simulink model "CMSD_Evaluation"  (R2024b)
settings: Solver=ode45  StartTime=0.0  StopTime=60  MaxStep=0.01  MinStep=0.01  RelTol=1e-3
undefined symbols (not defined in the file or in its folder): ref_seed
libraries: simulink x1, rllib x1
settings Model: Creator=minhh  LastModifiedBy=minhh
settings SolverCC: InitialStep=0.01

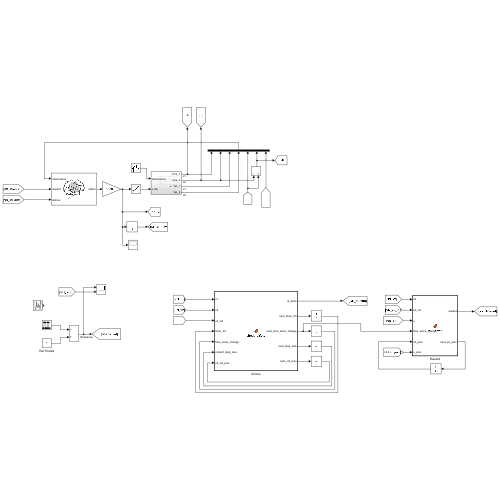
[thumbnail: Simulink's stored preview of the top-level diagram]
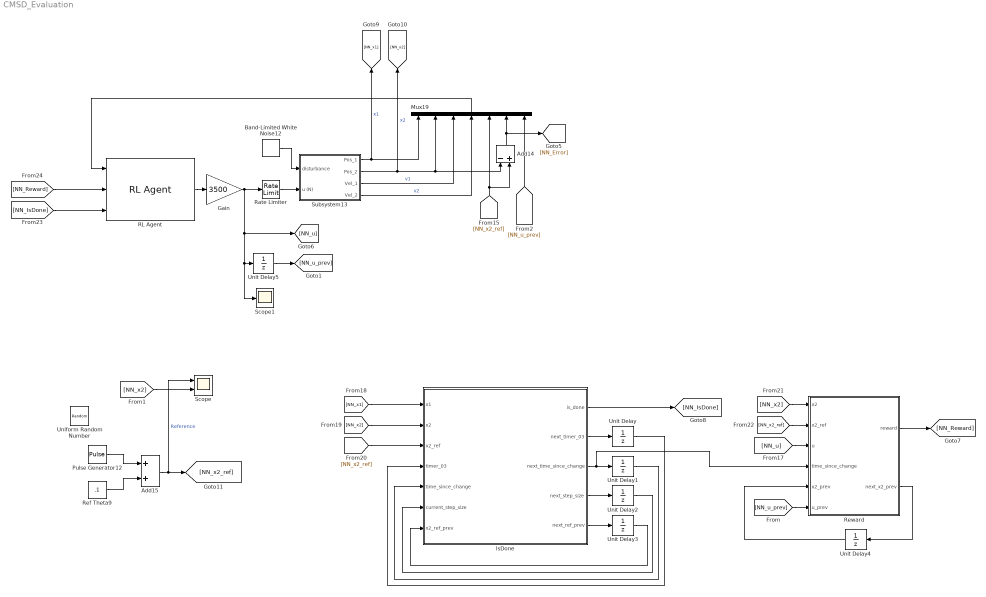
== system CMSD_Evaluation ==
  Add14 : Sum  Inputs=-+
  Add15 : Sum
  Band-Limited White Noise12 : simulink/Sources/Band-Limited White Noise  Cov=[200]  Ts=0.01  seed=[23341]
  Gain : Gain  Gain=3500
  IsDone : MATLAB Function  TreatAsAtomicUnit=on
  Mux19 : Mux  Inputs=7
  Pulse Generator12 : DiscretePulseGenerator  Amplitude=0.3  Period=10000  PulseWidth=2000  PhaseDelay=2000  SampleTime=0.01
  RL Agent : rllib/RL Agent  Agent=agentObj  ExternalActionAsInput=off  ProvideLastAction=off  ProvideCumRwd=off  TreatAsDirectFeedthrough=on  UseStrictObservationDataTypes=off
  Rate Limiter : RateLimiter  RisingSlewLimit=25000  FallingSlewLimit=-25000  SampleTimeMode=inherited
  Ref Theta9 : Constant  Value=.1  SampleTime=0.01
  Reward : MATLAB Function  TreatAsAtomicUnit=on
  Scope : Scope  NumInputPorts=2
  Scope1 : Scope
  Subsystem13 : Subsystem
  Uniform Random Number : UniformRandomNumber  Minimum=-0.2  Maximum=0.5  Seed=ref_seed  SampleTime=8
  Unit Delay{,1..5} (6 alike) : UnitDelay  SampleTime=0.01  HasFrameUpgradeWarning=on
  wires:
  [NN_IsDone] -> RL Agent/3
  [NN_x2] -> Reward/1(x2)
  IsDone/1(is_done) -> [NN_IsDone]
  Unit Delay3/1 -> IsDone/7(x2_ref_prev)
  Rate Limiter/1 -> Subsystem13/2(u (N))
  [NN_x2_ref] -> Mux19/5, Add14/2
  Unit Delay2/1 -> IsDone/6(current_step_size)
  IsDone/5(next_ref_prev) -> Unit Delay3/1
  [NN_x2_ref] -> IsDone/3(x2_ref)
  IsDone/2(next_timer_03) -> Unit Delay/1
  IsDone/3(next_time_since_change) -> Reward/4(time_since_change), Unit Delay1/1
  Unit Delay4/1 -> Reward/5(x2_prev)
  [NN_x2] -> IsDone/2(x2)
  Band-Limited White Noise12/1 -> Subsystem13/1(disturbance)
  Subsystem13/2(Pos_2) -> Add14/1, Mux19/2, [NN_x2]  "x2"
  [NN_u] -> Reward/3(u)
  IsDone/4(next_step_size) -> Unit Delay2/1
  Subsystem13/3(Vel_1) -> Mux19/3  "v1"
  [NN_Reward] -> RL Agent/2
  Reward/1(reward) -> [NN_Reward]
  [NN_x1] -> IsDone/1(x1)
  Unit Delay/1 -> IsDone/4(timer_03)
  Subsystem13/4(Vel_2) -> Mux19/4  "v2"
  [NN_x2_ref] -> Reward/2(x2_ref)
  Unit Delay1/1 -> IsDone/5(time_since_change)
  Gain/1 -> Scope1/1, Unit Delay5/1, [NN_u], Rate Limiter/1
  Reward/2(next_x2_prev) -> Unit Delay4/1
  Mux19/1 -> RL Agent/1
  Add14/1 -> [NN_Error], Mux19/6
  [NN_u_prev] -> Reward/6(u_prev)
  Unit Delay5/1 -> [NN_u_prev]
  Subsystem13/1(Pos_1) -> Mux19/1, [NN_x1]  "x1"
  RL Agent/1 -> Gain/1
  Pulse Generator12/1 -> Add15/1
  Ref Theta9/1 -> Add15/2
  [NN_x2] -> Scope/2
  Add15/1 -> Scope/1, [NN_x2_ref]  "Reference"
  [NN_u_prev] -> Mux19/7

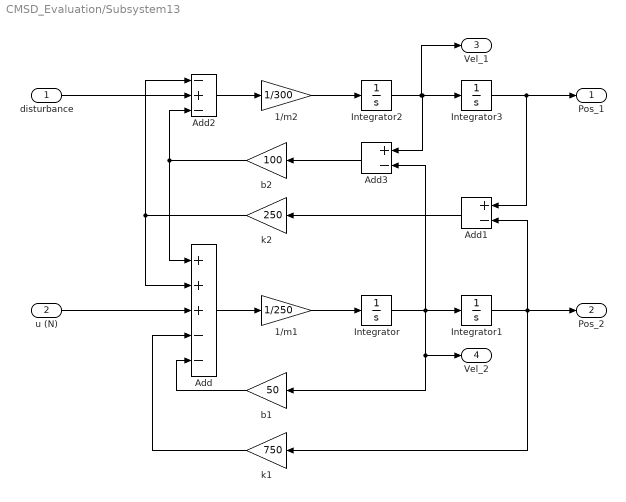
== system CMSD_Evaluation/Subsystem13 ==
  disturbance : Inport
  u (N) : Inport  Port=2
  1/m1 : Gain  Gain=1/250
  1/m2 : Gain  Gain=1/300
  Add : Sum  Inputs=+++--
  Add1 : Sum  Inputs=+-
  Add2 : Sum  Inputs=-+-
  Add3 : Sum  Inputs=+-
  Integrator{,1..3} (4 alike) : Integrator
  b1 : Gain  Gain=50
  b2 : Gain  Gain=100
  k1 : Gain  Gain=750
  k2 : Gain  Gain=250
  Pos_1 : Outport
  Pos_2 : Outport  Port=2
  Vel_1 : Outport  Port=3
  Vel_2 : Outport  Port=4
  wires:
  Add/1 -> 1/m1/1
  1/m1/1 -> Integrator/1
  Integrator/1 -> Add3/2, Integrator1/1, b1/1, Vel_2/1
  Integrator1/1 -> k1/1, Pos_2/1, Add1/2
  Add2/1 -> 1/m2/1
  1/m2/1 -> Integrator2/1
  Integrator2/1 -> Vel_1/1, Add3/1, Integrator3/1
  Add3/1 -> b2/1
  b2/1 -> Add2/3, Add/1
  Add1/1 -> k2/1
  Integrator3/1 -> Pos_1/1, Add1/1
  u (N)/1 -> Add/3
  b1/1 -> Add/5
  k1/1 -> Add/4
  k2/1 -> Add2/1, Add/2
  disturbance/1 -> Add2/2

== matlab function CMSD_Evaluation/Reward ==
  data: x2 input; x2_ref input; u input; reward output; time_since_change input; x2_prev input; next_x2_prev output; u_prev input
function [reward, next_x2_prev] = calc_reward(x2, x2_ref, u, time_since_change, x2_prev, u_prev)
    
    % --- ENFORCE STRICT DATA TYPES FOR COMPILER ---
    reward = double(0.1); 
    next_x2_prev = double(x2); 
    
    x2_error = double(abs(x2_ref - x2));
    delta_x2 = double(abs(x2 - x2_prev));
    delta_u  = double(abs(u - u_prev));
    
    % --- 1. TIGHT BOUNDARY BLEED (0.0050m) ---
    reward = double(reward - (10.0 * x2_error^2)); 
    
    if x2_error > 0.0050
        reward = double(reward - 1.0); 
    else
        reward = double(reward + 2.0); 
    end
    
    % --- 2. SMC ROBUSTNESS (Settle-Time Grace Period) ---
    if time_since_change > 1.0
        if delta_x2 > 0.005
            reward = double(reward - 5.0); 
        end
    end
    
    % --- 3. ENERGY EFFICIENCY ---
    reward = double(reward - 0.5 * ((u / 3500.0)^2));
    
    % --- 4. HARDWARE LIMIT PENALTY (250N/step) ---
    if delta_u > 500.0
        violation = double(delta_u - 500.0);
        reward = double(reward - (violation^2)); 
    end

    % --- THE ANTI-SUICIDE PATCH ---
    % If the AI violently jerks the motor and breaks the x1 limit, 
    % it receives a penalty so massive it will never do it again.
    if abs(x1) > 0.65
        reward = double(reward - 6000.0);
    end
    
end

== matlab function CMSD_Evaluation/IsDone ==
  data: x1 input; is_done output; x2 input; x2_ref input; next_timer_03 output; timer_03 input; time_since_change input; current_step_size input; x2_ref_prev input; next_time_since_change output; next_step_size output; next_ref_prev output
function [is_done, next_timer_03, next_time_since_change, next_step_size, next_ref_prev] = check_safety(x1, x2, x2_ref, timer_03, time_since_change, current_step_size, x2_ref_prev)
    
    % --- ENFORCE STRICT DATA TYPES FOR THE COMPILER ---
    is_done = double(0); % <--- Changed to double(0) instead of false
    next_timer_03 = double(timer_03);
    next_time_since_change = double(time_since_change);
    next_step_size = double(current_step_size);
    next_ref_prev = double(x2_ref_prev);
    
    dt = double(0.01); 
    x2_error = double(x2_ref - x2);
    
    % --- 1. DETECT A REFERENCE CHANGE ---
    if abs(x2_ref - x2_ref_prev) > 0.001
        next_time_since_change = double(0.0);
        next_step_size = double(abs(x2_ref - x2_ref_prev));
    else
        next_time_since_change = double(time_since_change + dt);
    end
    next_ref_prev = double(x2_ref);
    
    % --- 2. DEATH CONDITIONS ---
    if abs(x1) > 0.65
        is_done = double(1); % <--- Changed to double(1) instead of true
    end
    
% --- RELAXED DEATH CONDITIONS FOR CURRICULUM LEARNING ---
    
    % Give it 3.0 seconds to fix a massive error instead of 0.75s
    if abs(x2_error) > 0.3
        next_timer_03 = double(timer_03 + dt);
    else
        next_timer_03 = double(0.0);
    end
    
    if next_timer_03 > 3.0
        is_done = double(1); 
    end
    
    % Give it a flat 5.0 seconds to settle, bypassing the 2.2x multiplier
    allowed_settle_time = double(5.0); 
    
    % Widen the survival boundary to 0.050m for early training
    if (next_time_since_change > allowed_settle_time) && (abs(x2_error) > 0.050) 
        is_done = double(1); 
    end
end
